simulink model "Y3Tiltrotor_sim3_IINDI_case2_1"  (R2025a)
settings: Solver=ode4  StartTime=0.0  StopTime=80  FixedStep=uavParam.sampleTime  RelTol=1e-3
PreLoadFcn:
  | filepath  = fileparts(get_param(bdroot, 'FileName'))
  | cd(filepath);
InitFcn:
  | Init_sim_IINDI_case2_1;
values from neighbouring files (symbols this model uses):
  a_HOD_p = 5    [Init_sim_IINDI_case2.m]    (also in Init_sim_IINDI_case2_1.m)
  a_HOD_q = 5    [Init_sim_IINDI_case2.m]    (also in Init_sim_IINDI_case2_1.m = 25)
  a_HOD_r = 5    [Init_sim_IINDI_case2.m]    (also in Init_sim_IINDI_case2_1.m)
  a_HOD_u = 5    [Init_sim_IINDI_case2.m]    (also in Init_sim_IINDI_case2_1.m = 15)
  a_HOD_v = 2    [Init_sim_IINDI_case2.m]    (also in Init_sim_IINDI_case2_1.m)
  a_HOD_w = 30    [Init_sim_IINDI_case2.m]    (also in Init_sim_IINDI_case2_1.m = 10)
  control = struct    [Init_sim_IINDI_case2.m]    (also in Init_sim_IINDI_case2_1.m)
  env = struct    [InitData.m]
  flightState = struct    [Init_sim_IINDI_case2.m]    (also in Init_sim_IINDI_case2_1.m)
  FWSpeed0 = 15    [Init_sim_IINDI_case2.m]    (also in Init_sim_IINDI_case2_1.m)
  k_lpf_p = 50    [Init_sim_IINDI_case2.m]    (also in Init_sim_IINDI_case2_1.m)
  k_lpf_q = 80    [Init_sim_IINDI_case2.m]    (also in Init_sim_IINDI_case2_1.m = 150)
  k_lpf_r = 100    [Init_sim_IINDI_case2.m]    (also in Init_sim_IINDI_case2_1.m)
  k_lpf_u = 8    [Init_sim_IINDI_case2.m]    (also in Init_sim_IINDI_case2_1.m)
  k_lpf_v = 1.5    [Init_sim_IINDI_case2.m]    (also in Init_sim_IINDI_case2_1.m)
  k_lpf_w = 50    [Init_sim_IINDI_case2.m]    (also in Init_sim_IINDI_case2_1.m)
  k_p = 5    [Init_sim_IINDI_case2.m]    (also in Init_sim_IINDI_case2_1.m)
  k_q = 12    [Init_sim_IINDI_case2.m]    (also in Init_sim_IINDI_case2_1.m)
  k_r = 0.1    [Init_sim_IINDI_case2.m]    (also in Init_sim_IINDI_case2_1.m)
  k_u = 0.2    [Init_sim_IINDI_case2.m]    (also in Init_sim_IINDI_case2_1.m = 1)
  k_v = 0.7    [Init_sim_IINDI_case2.m]    (also in Init_sim_IINDI_case2_1.m = 0.2)
  k_w = 2    [Init_sim_IINDI_case2.m]    (also in Init_sim_IINDI_case2_1.m)
  l_p = 30    [Init_sim_IINDI_case2.m]    (also in Init_sim_IINDI_case2_1.m)
  l_q = 15    [Init_sim_IINDI_case2.m]    (also in Init_sim_IINDI_case2_1.m)
  l_r = 25    [Init_sim_IINDI_case2.m]    (also in Init_sim_IINDI_case2_1.m)
  l_u = 1    [Init_sim_IINDI_case2.m]    (also in Init_sim_IINDI_case2_1.m = 0.8)
  l_v = 1.2    [Init_sim_IINDI_case2.m]    (also in Init_sim_IINDI_case2_1.m)
  l_w = 1    [Init_sim_IINDI_case2.m]    (also in Init_sim_IINDI_case2_1.m)
  lamda_p = 10    [Init_sim_IINDI_case2.m]    (also in Init_sim_IINDI_case2_1.m)
  lamda_q = 5    [Init_sim_IINDI_case2.m]    (also in Init_sim_IINDI_case2_1.m)
  lamda_r = 1    [Init_sim_IINDI_case2.m]    (also in Init_sim_IINDI_case2_1.m)
  lamda_u = 1    [Init_sim_IINDI_case2.m]    (also in Init_sim_IINDI_case2_1.m)
  lamda_v = 0.15    [Init_sim_IINDI_case2.m]    (also in Init_sim_IINDI_case2_1.m)
  lamda_w = 1    [Init_sim_IINDI_case2.m]    (also in Init_sim_IINDI_case2_1.m)
  uavParam = struct    [InitData.m]
undefined symbols (not defined in the file or in its folder): a_HOD, a_HOD_uvw, ControlSampleTime, F, Light, MIL, Newton, Raphson
libraries: slpidlib x31, SignalEditorBlockLib x15, simulink x3, aerolibtransform2 x3, sharedtransform x3, robotcorelib x3, matrix_library x3, aerolibasang x2, aerolibutil x2, aerolibwind2 x2, shared6dof x1, aerolibatmos2 x1
(part 2 of 8)

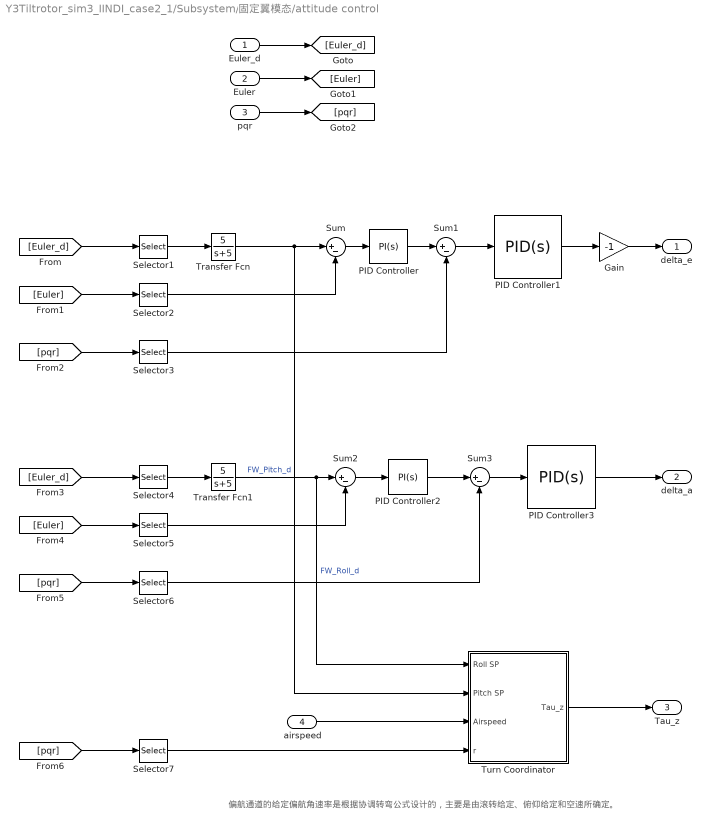
== system Y3Tiltrotor_sim3_IINDI_case2_1/Subsystem/固定翼模态/attitude control ==
  note: 偏航通道的给定偏航角速率是根据协调转弯公式设计的，主要是由滚转给定、俯仰给定和空速所确定。
  Euler_d : Inport
  Euler : Inport  Port=2
  pqr : Inport  Port=3
  airspeed : Inport  Port=4
  Gain : Gain  Gain=-1
  PID Controller : slpidlib/PID Controller  Controller=PI  Form=Parallel  TimeDomain=Continuous-time  UseExternalTs=off  SampleTime=ControlSampleTime  IntegratorMethod=Forward Euler  FilterMethod=Forward Euler  ControllerParametersSource=internal  P=control.FW.pitch_P  I=control.FW.pitch_I  UseKiTs=off  D=0  UseExternalDerivativeSource=off  N=100  UseFilter=on  TunerSelectOption=Transfer Function Based (PID Tuner App)  InitialConditionSource=internal  InitialConditionForIntegrator=0  InitialConditionForFilter=0  DifferentiatorICPrevScaledInput=0  ExternalReset=none  TrackingMode=off  Kt=1  LimitOutput=on  SatLimitsSource=internal  UpperSaturationLimit=control.maxPitchRate  LowerSaturationLimit=control.minPitchRate  LinearizeAsGain=on  AntiWindupMode=clamping  Kb=1  LimitIntegrator=off  UpperIntegratorSaturationLimit=inf  LowerIntegratorSaturationLimit=-inf  POutMin=[]  POutMax=[]  IOutMin=[]  IOutMax=[]  DOutMin=[]  DOutMax=[]  NOutMin=[]  NOutMax=[]  SumOutMin=[]  SumOutMax=[]  SaturationOutMin=[]  SaturationOutMax=[]  PParamMin=[]  PParamMax=[]  IParamMin=[]  IParamMax=[]  DParamMin=[]  DParamMax=[]  NParamMin=[]  NParamMax=[]  KbParamMin=[]  KbParamMax=[]  KtParamMin=[]  KtParamMax=[]  KbOutMin=[]  KbOutMax=[]  KtOutMin=[]  KtOutMax=[]  IntegratorOutMin=[]  IntegratorOutMax=[]  FilterOutMin=[]  FilterOutMax=[]  SumI1OutMin=[]  SumI1OutMax=[]  SumI2OutMin=[]  SumI2OutMax=[]  SumI3OutMin=[]  SumI3OutMax=[]  SumI4OutMin=[]  SumI4OutMax=[]  SumDOutMin=[]  SumDOutMax=[]  DifferentiatorOutMin=[]  DifferentiatorOutMax=[]  FilterDiffOutCoefMin=[]  FilterDiffOutCoefMax=[]  ReciprocalOutMin=[]  ReciprocalOutMax=[]  SumDenOutMin=[]  SumDenOutMax=[]  SumNumOutMin=[]  SumNumOutMax=[]  DivideOutMin=[]  DivideOutMax=[]  UdiffTsProdOutMin=[]  UdiffTsProdOutMax=[]  NTsProdOutMin=[]  NTsProdOutMax=[]  UintegralTsProdOutMin=[]  UintegralTsProdOutMax=[]  UngainTsProdOutMin=[]  UngainTsProdOutMax=[]  ClampingZeroOutDataTypeStr=Inherit: Inherit via back propagation  ClampingZeroOutMin=[]  ClampingZeroOutMax=[]  FilterDenConstantOutDataTypeStr=Inherit: Inherit via back propagation  FilterDenConstantOutMin=[]  FilterDenConstantOutMax=[]  PCopyOutDataTypeStr=Inherit: Inherit via back propagation  PCopyOutMin=[]  PCopyOutMax=[]  NCopyOutDataTypeStr=Inherit: Inherit via back propagation  NCopyOutMin=[]  NCopyOutMax=[]  IntegratorContinuousStateAttributes=''  IntegratorStateMustResolveToSignalObject=off  IntegratorRTWStateStorageClass=Auto  FilterContinuousStateAttributes=''  FilterStateMustResolveToSignalObject=off  FilterRTWStateStorageClass=Auto  ParallelPVariant=InternalParameters  IdealPVariant=Disabled  IVariant=InternalParameters  DVariant=Disabled  IntegratorVariant=Continuous  SatVariant=Enabled  AWVariant=ContClampingParallel  PCopyVariant=Disabled  TRVariant=Disabled  FdbkBlocksVariant=Forward  IdealPFdbkVariant=Disabled  SatFdbkVariant=Disabled  DerivativeFilterVariant=Disabled  NVariant=Disabled  NCopyVariant=Disabled_SignalSpec  FilterICVariant=Disabled  IntegratorICVariant=InternalICs  ExternalResetVariant=Disabled  TRSumVariant=Passthrough  SumFdbkVariant=Disabled  SumVariant=Sum_PI  TsampFilterVariant=InternalTs  TsampNgainVariant=Passthrough  TsampIntegralVariant=Disabled_SignalSpec  ExternalSaturationOutDataTypeStr=Inherit: Same as second input  DerivativeSourceVariant=Disabled  PreIntVariant=InternalPreInt
  PID Controller1 : slpidlib/PID Controller  Controller=PID  Form=Parallel  TimeDomain=Continuous-time  UseExternalTs=off  SampleTime=ControlSampleTime  IntegratorMethod=Forward Euler  FilterMethod=Forward Euler  ControllerParametersSource=internal  P=control.FW.pitchRate_P  I=control.FW.pitchRate_I  UseKiTs=off  D=control.FW.pitchRate_D  UseExternalDerivativeSource=off  N=10  UseFilter=on  TunerSelectOption=Transfer Function Based (PID Tuner App)  InitialConditionSource=internal  InitialConditionForIntegrator=0  InitialConditionForFilter=0  DifferentiatorICPrevScaledInput=0  ExternalReset=none  TrackingMode=off  Kt=1  LimitOutput=on  SatLimitsSource=internal  UpperSaturationLimit=pi/2  LowerSaturationLimit=-pi/2  LinearizeAsGain=on  AntiWindupMode=clamping  Kb=1  LimitIntegrator=off  UpperIntegratorSaturationLimit=inf  LowerIntegratorSaturationLimit=-inf  POutMin=[]  POutMax=[]  IOutMin=[]  IOutMax=[]  DOutMin=[]  DOutMax=[]  NOutMin=[]  NOutMax=[]  SumOutMin=[]  SumOutMax=[]  SaturationOutMin=[]  SaturationOutMax=[]  PParamMin=[]  PParamMax=[]  IParamMin=[]  IParamMax=[]  DParamMin=[]  DParamMax=[]  NParamMin=[]  NParamMax=[]  KbParamMin=[]  KbParamMax=[]  KtParamMin=[]  KtParamMax=[]  KbOutMin=[]  KbOutMax=[]  KtOutMin=[]  KtOutMax=[]  IntegratorOutMin=[]  IntegratorOutMax=[]  FilterOutMin=[]  FilterOutMax=[]  SumI1OutMin=[]  SumI1OutMax=[]  SumI2OutMin=[]  SumI2OutMax=[]  SumI3OutMin=[]  SumI3OutMax=[]  SumI4OutMin=[]  SumI4OutMax=[]  SumDOutMin=[]  SumDOutMax=[]  DifferentiatorOutMin=[]  DifferentiatorOutMax=[]  FilterDiffOutCoefMin=[]  FilterDiffOutCoefMax=[]  ReciprocalOutMin=[]  ReciprocalOutMax=[]  SumDenOutMin=[]  SumDenOutMax=[]  SumNumOutMin=[]  SumNumOutMax=[]  DivideOutMin=[]  DivideOutMax=[]  UdiffTsProdOutMin=[]  UdiffTsProdOutMax=[]  NTsProdOutMin=[]  NTsProdOutMax=[]  UintegralTsProdOutMin=[]  UintegralTsProdOutMax=[]  UngainTsProdOutMin=[]  UngainTsProdOutMax=[]  ClampingZeroOutDataTypeStr=Inherit: Inherit via back propagation  ClampingZeroOutMin=[]  ClampingZeroOutMax=[]  FilterDenConstantOutDataTypeStr=Inherit: Inherit via back propagation  FilterDenConstantOutMin=[]  FilterDenConstantOutMax=[]  PCopyOutDataTypeStr=Inherit: Inherit via back propagation  PCopyOutMin=[]  PCopyOutMax=[]  NCopyOutDataTypeStr=Inherit: Inherit via back propagation  NCopyOutMin=[]  NCopyOutMax=[]  IntegratorContinuousStateAttributes=''  IntegratorStateMustResolveToSignalObject=off  IntegratorRTWStateStorageClass=Auto  FilterContinuousStateAttributes=''  FilterStateMustResolveToSignalObject=off  FilterRTWStateStorageClass=Auto  ParallelPVariant=InternalParameters  IdealPVariant=Disabled  IVariant=InternalParameters  DVariant=InternalParameters  IntegratorVariant=Continuous  SatVariant=Enabled  AWVariant=ContClampingParallel  PCopyVariant=Disabled  TRVariant=Disabled  FdbkBlocksVariant=Forward  IdealPFdbkVariant=Disabled  SatFdbkVariant=Disabled  DerivativeFilterVariant=ContFilter  NVariant=InternalParameters  NCopyVariant=Disabled  FilterICVariant=InternalICsFilter  IntegratorICVariant=InternalICs  ExternalResetVariant=Disabled  TRSumVariant=Passthrough  SumFdbkVariant=Disabled  SumVariant=Sum_PID  TsampFilterVariant=InternalTs  TsampNgainVariant=Passthrough  TsampIntegralVariant=Disabled_SignalSpec  ExternalSaturationOutDataTypeStr=Inherit: Same as second input  DerivativeSourceVariant=ErrorSignal  PreIntVariant=InternalPreInt
  PID Controller2 : slpidlib/PID Controller  Controller=PI  Form=Parallel  TimeDomain=Continuous-time  UseExternalTs=off  SampleTime=ControlSampleTime  IntegratorMethod=Forward Euler  FilterMethod=Forward Euler  ControllerParametersSource=internal  P=control.FW.roll_P  I=control.FW.roll_I  UseKiTs=off  D=0  UseExternalDerivativeSource=off  N=100  UseFilter=on  TunerSelectOption=Transfer Function Based (PID Tuner App)  InitialConditionSource=internal  InitialConditionForIntegrator=0  InitialConditionForFilter=0  DifferentiatorICPrevScaledInput=0  ExternalReset=none  TrackingMode=off  Kt=1  LimitOutput=on  SatLimitsSource=internal  UpperSaturationLimit=control.maxRollRate  LowerSaturationLimit=control.minRollRate  LinearizeAsGain=on  AntiWindupMode=clamping  Kb=1  LimitIntegrator=off  UpperIntegratorSaturationLimit=inf  LowerIntegratorSaturationLimit=-inf  POutMin=[]  POutMax=[]  IOutMin=[]  IOutMax=[]  DOutMin=[]  DOutMax=[]  NOutMin=[]  NOutMax=[]  SumOutMin=[]  SumOutMax=[]  SaturationOutMin=[]  SaturationOutMax=[]  PParamMin=[]  PParamMax=[]  IParamMin=[]  IParamMax=[]  DParamMin=[]  DParamMax=[]  NParamMin=[]  NParamMax=[]  KbParamMin=[]  KbParamMax=[]  KtParamMin=[]  KtParamMax=[]  KbOutMin=[]  KbOutMax=[]  KtOutMin=[]  KtOutMax=[]  IntegratorOutMin=[]  IntegratorOutMax=[]  FilterOutMin=[]  FilterOutMax=[]  SumI1OutMin=[]  SumI1OutMax=[]  SumI2OutMin=[]  SumI2OutMax=[]  SumI3OutMin=[]  SumI3OutMax=[]  SumI4OutMin=[]  SumI4OutMax=[]  SumDOutMin=[]  SumDOutMax=[]  DifferentiatorOutMin=[]  DifferentiatorOutMax=[]  FilterDiffOutCoefMin=[]  FilterDiffOutCoefMax=[]  ReciprocalOutMin=[]  ReciprocalOutMax=[]  SumDenOutMin=[]  SumDenOutMax=[]  SumNumOutMin=[]  SumNumOutMax=[]  DivideOutMin=[]  DivideOutMax=[]  UdiffTsProdOutMin=[]  UdiffTsProdOutMax=[]  NTsProdOutMin=[]  NTsProdOutMax=[]  UintegralTsProdOutMin=[]  UintegralTsProdOutMax=[]  UngainTsProdOutMin=[]  UngainTsProdOutMax=[]  ClampingZeroOutDataTypeStr=Inherit: Inherit via back propagation  ClampingZeroOutMin=[]  ClampingZeroOutMax=[]  FilterDenConstantOutDataTypeStr=Inherit: Inherit via back propagation  FilterDenConstantOutMin=[]  FilterDenConstantOutMax=[]  PCopyOutDataTypeStr=Inherit: Inherit via back propagation  PCopyOutMin=[]  PCopyOutMax=[]  NCopyOutDataTypeStr=Inherit: Inherit via back propagation  NCopyOutMin=[]  NCopyOutMax=[]  IntegratorContinuousStateAttributes=''  IntegratorStateMustResolveToSignalObject=off  IntegratorRTWStateStorageClass=Auto  FilterContinuousStateAttributes=''  FilterStateMustResolveToSignalObject=off  FilterRTWStateStorageClass=Auto  ParallelPVariant=InternalParameters  IdealPVariant=Disabled  IVariant=InternalParameters  DVariant=Disabled  IntegratorVariant=Continuous  SatVariant=Enabled  AWVariant=ContClampingParallel  PCopyVariant=Disabled  TRVariant=Disabled  FdbkBlocksVariant=Forward  IdealPFdbkVariant=Disabled  SatFdbkVariant=Disabled  DerivativeFilterVariant=Disabled  NVariant=Disabled  NCopyVariant=Disabled_SignalSpec  FilterICVariant=Disabled  IntegratorICVariant=InternalICs  ExternalResetVariant=Disabled  TRSumVariant=Passthrough  SumFdbkVariant=Disabled  SumVariant=Sum_PI  TsampFilterVariant=InternalTs  TsampNgainVariant=Passthrough  TsampIntegralVariant=Disabled_SignalSpec  ExternalSaturationOutDataTypeStr=Inherit: Same as second input  DerivativeSourceVariant=Disabled  PreIntVariant=InternalPreInt
  PID Controller3 : slpidlib/PID Controller  Controller=PID  Form=Parallel  TimeDomain=Continuous-time  UseExternalTs=off  SampleTime=ControlSampleTime  IntegratorMethod=Forward Euler  FilterMethod=Forward Euler  ControllerParametersSource=internal  P=control.FW.rollRate_P  I=control.FW.rollRate_I  UseKiTs=off  D=control.FW.rollRate_D  UseExternalDerivativeSource=off  N=10  UseFilter=on  TunerSelectOption=Transfer Function Based (PID Tuner App)  InitialConditionSource=internal  InitialConditionForIntegrator=0  InitialConditionForFilter=0  DifferentiatorICPrevScaledInput=0  ExternalReset=none  TrackingMode=off  Kt=1  LimitOutput=on  SatLimitsSource=internal  UpperSaturationLimit=pi/2  LowerSaturationLimit=-pi/2  LinearizeAsGain=on  AntiWindupMode=clamping  Kb=1  LimitIntegrator=off  UpperIntegratorSaturationLimit=inf  LowerIntegratorSaturationLimit=-inf  POutMin=[]  POutMax=[]  IOutMin=[]  IOutMax=[]  DOutMin=[]  DOutMax=[]  NOutMin=[]  NOutMax=[]  SumOutMin=[]  SumOutMax=[]  SaturationOutMin=[]  SaturationOutMax=[]  PParamMin=[]  PParamMax=[]  IParamMin=[]  IParamMax=[]  DParamMin=[]  DParamMax=[]  NParamMin=[]  NParamMax=[]  KbParamMin=[]  KbParamMax=[]  KtParamMin=[]  KtParamMax=[]  KbOutMin=[]  KbOutMax=[]  KtOutMin=[]  KtOutMax=[]  IntegratorOutMin=[]  IntegratorOutMax=[]  FilterOutMin=[]  FilterOutMax=[]  SumI1OutMin=[]  SumI1OutMax=[]  SumI2OutMin=[]  SumI2OutMax=[]  SumI3OutMin=[]  SumI3OutMax=[]  SumI4OutMin=[]  SumI4OutMax=[]  SumDOutMin=[]  SumDOutMax=[]  DifferentiatorOutMin=[]  DifferentiatorOutMax=[]  FilterDiffOutCoefMin=[]  FilterDiffOutCoefMax=[]  ReciprocalOutMin=[]  ReciprocalOutMax=[]  SumDenOutMin=[]  SumDenOutMax=[]  SumNumOutMin=[]  SumNumOutMax=[]  DivideOutMin=[]  DivideOutMax=[]  UdiffTsProdOutMin=[]  UdiffTsProdOutMax=[]  NTsProdOutMin=[]  NTsProdOutMax=[]  UintegralTsProdOutMin=[]  UintegralTsProdOutMax=[]  UngainTsProdOutMin=[]  UngainTsProdOutMax=[]  ClampingZeroOutDataTypeStr=Inherit: Inherit via back propagation  ClampingZeroOutMin=[]  ClampingZeroOutMax=[]  FilterDenConstantOutDataTypeStr=Inherit: Inherit via back propagation  FilterDenConstantOutMin=[]  FilterDenConstantOutMax=[]  PCopyOutDataTypeStr=Inherit: Inherit via back propagation  PCopyOutMin=[]  PCopyOutMax=[]  NCopyOutDataTypeStr=Inherit: Inherit via back propagation  NCopyOutMin=[]  NCopyOutMax=[]  IntegratorContinuousStateAttributes=''  IntegratorStateMustResolveToSignalObject=off  IntegratorRTWStateStorageClass=Auto  FilterContinuousStateAttributes=''  FilterStateMustResolveToSignalObject=off  FilterRTWStateStorageClass=Auto  ParallelPVariant=InternalParameters  IdealPVariant=Disabled  IVariant=InternalParameters  DVariant=InternalParameters  IntegratorVariant=Continuous  SatVariant=Enabled  AWVariant=ContClampingParallel  PCopyVariant=Disabled  TRVariant=Disabled  FdbkBlocksVariant=Forward  IdealPFdbkVariant=Disabled  SatFdbkVariant=Disabled  DerivativeFilterVariant=ContFilter  NVariant=InternalParameters  NCopyVariant=Disabled  FilterICVariant=InternalICsFilter  IntegratorICVariant=InternalICs  ExternalResetVariant=Disabled  TRSumVariant=Passthrough  SumFdbkVariant=Disabled  SumVariant=Sum_PID  TsampFilterVariant=InternalTs  TsampNgainVariant=Passthrough  TsampIntegralVariant=Disabled_SignalSpec  ExternalSaturationOutDataTypeStr=Inherit: Same as second input  DerivativeSourceVariant=ErrorSignal  PreIntVariant=InternalPreInt
  Selector1 : Selector  InputPortWidth=3  IndexOptions=Index vector (dialog)  Indices=2  OutputSizes=1
  Selector2 : Selector  InputPortWidth=3  IndexOptions=Index vector (dialog)  Indices=2  OutputSizes=1
  Selector3 : Selector  InputPortWidth=3  IndexOptions=Index vector (dialog)  Indices=2  OutputSizes=1
  Selector4 : Selector  InputPortWidth=3  IndexOptions=Index vector (dialog)  Indices=1  OutputSizes=1
  Selector5 : Selector  InputPortWidth=3  IndexOptions=Index vector (dialog)  Indices=1  OutputSizes=1
  Selector6 : Selector  InputPortWidth=3  IndexOptions=Index vector (dialog)  Indices=1  OutputSizes=1
  Selector7 : Selector  InputPortWidth=3  IndexOptions=Index vector (dialog)  Indices=3  OutputSizes=1
  Sum{,1..3} (4 alike) : Sum  Inputs=|+-
  Transfer Fcn : TransferFcn  Numerator=[5]  Denominator=[1 5]
  Transfer Fcn1 : TransferFcn  Numerator=[5]  Denominator=[1 5]
  Turn Coordinator : Subsystem
  delta_e : Outport
  delta_a : Outport  Port=2
  Tau_z : Outport  Port=3
  wires:
  Selector2/1 -> Sum/2
  Sum/1 -> PID Controller/1
  Selector3/1 -> Sum1/2
  Sum1/1 -> PID Controller1/1
  PID Controller1/1 -> Gain/1
  Selector1/1 -> Transfer Fcn/1
  PID Controller/1 -> Sum1/1
  Euler_d/1 -> [Euler_d]
  Euler/1 -> [Euler]
  pqr/1 -> [pqr]
  [Euler_d] -> Selector1/1
  [Euler] -> Selector2/1
  [pqr] -> Selector3/1
  [pqr] -> Selector6/1
  [Euler_d] -> Selector4/1
  [Euler] -> Selector5/1
  Transfer Fcn1/1 -> Turn Coordinator/1(Roll SP), Sum2/1  "FW_Roll_d"
  Selector5/1 -> Sum2/2
  Sum2/1 -> PID Controller2/1
  Sum3/1 -> PID Controller3/1
  Selector6/1 -> Sum3/2
  PID Controller2/1 -> Sum3/1
  Selector4/1 -> Transfer Fcn1/1
  airspeed/1 -> Turn Coordinator/3(Airspeed)
  [pqr] -> Selector7/1
  Selector7/1 -> Turn Coordinator/4(r)
  Transfer Fcn/1 -> Turn Coordinator/2(Pitch SP), Sum/1  "FW_Pitch_d"
  Gain/1 -> delta_e/1
  PID Controller3/1 -> delta_a/1
  Turn Coordinator/1(Tau_z) -> Tau_z/1

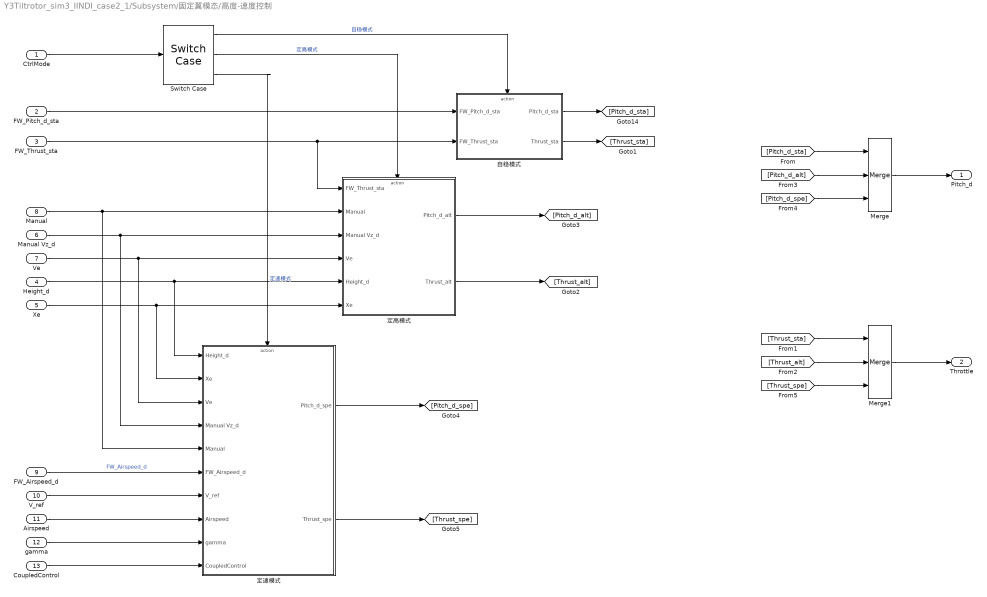
== system Y3Tiltrotor_sim3_IINDI_case2_1/Subsystem/固定翼模态/高度-速度控制 ==
  CtrlMode : Inport
  FW_Pitch_d_sta : Inport  Port=2
  FW_Thrust_sta : Inport  Port=3
  Height_d : Inport  Port=4
  Xe : Inport  Port=5
  Manual Vz_d : Inport  Port=6
  Ve : Inport  Port=7
  Manual : Inport  Port=8
  FW_Airspeed_d : Inport  Port=9
  V_ref : Inport  Port=10
  Airspeed : Inport  Port=11
  gamma : Inport  Port=12
  CoupledControl : Inport  Port=13
  Merge : Merge  Inputs=3
  Merge1 : Merge  Inputs=3
  Switch Case : SwitchCase  CaseConditions={0,1,2}  ShowDefaultCase=off
  定速模式 : Subsystem
  定高模式 : Subsystem
  自稳模式 : Subsystem
  Pitch_d : Outport
  Throttle : Outport  Port=2
  wires:
  Switch Case/3 -> 定速模式/Action  "定速模式"
  Switch Case/1 -> 自稳模式/Action  "自稳模式"
  Switch Case/2 -> 定高模式/Action  "定高模式"
  CtrlMode/1 -> Switch Case/1
  FW_Pitch_d_sta/1 -> 自稳模式/1(FW_Pitch_d_sta)
  FW_Thrust_sta/1 -> 定高模式/1(FW_Thrust_sta), 自稳模式/2(FW_Thrust_sta)
  Merge/1 -> Pitch_d/1
  自稳模式/1(Pitch_d_sta) -> [Pitch_d_sta]
  自稳模式/2(Thrust_sta) -> [Thrust_sta]
  [Pitch_d_sta] -> Merge/1
  [Thrust_sta] -> Merge1/1
  定高模式/2(Thrust_alt) -> [Thrust_alt]
  [Thrust_alt] -> Merge1/2
  定高模式/1(Pitch_d_alt) -> [Pitch_d_alt]
  Xe/1 -> 定速模式/2(Xe), 定高模式/6(Xe)
  Manual Vz_d/1 -> 定速模式/4(Manual Vz_d), 定高模式/3(Manual Vz_d)
  Ve/1 -> 定速模式/3(Ve), 定高模式/4(Ve)
  Manual/1 -> 定高模式/2(Manual), 定速模式/5(Manual)
  定速模式/1(Pitch_d_spe) -> [Pitch_d_spe]
  定速模式/2(Thrust_spe) -> [Thrust_spe]
  [Pitch_d_spe] -> Merge/3
  [Thrust_spe] -> Merge1/3
  Height_d/1 -> 定速模式/1(Height_d), 定高模式/5(Height_d)
  FW_Airspeed_d/1 -> 定速模式/6(FW_Airspeed_d)  "FW_Airspeed_d"
  Airspeed/1 -> 定速模式/8(Airspeed)
  gamma/1 -> 定速模式/9(gamma)
  CoupledControl/1 -> 定速模式/10(CoupledControl)
  [Pitch_d_alt] -> Merge/2
  V_ref/1 -> 定速模式/7(V_ref)
  Merge1/1 -> Throttle/1

== system Y3Tiltrotor_sim3_IINDI_case2_1/Subsystem/多旋翼模态/InputConditioning_stablelize ==
  Ch1 : Inport
  Ch2 : Inport  Port=2
  Ch3 : Inport  Port=3
  Ch4 : Inport  Port=4
  Manual : Inport  Port=5
  theta_ref : Inport  Port=6
  Constant : Constant
  Constant1 : Constant  Value=0
  Gain : Gain  Gain=0.5
  Gain13 : Gain  Gain=control.maxPitch
  Gain14 : Gain  Gain=control.maxRoll
  Gain15 : Gain  Gain=control.maxYawRate
  Gain16 : Gain  Gain=3
  Gain2 : Gain  Gain=pi/180
  Saturation{1,7..9} (4 alike) : Saturate  UpperLimit=1  LowerLimit=-1
  Saturation10 : Saturate  UpperLimit=1  LowerLimit=0
  Saturation4 : Saturate  UpperLimit=3  LowerLimit=0
  Sum : Sum  Inputs=|++
  Switch : Switch  Criteria=u2 > Threshold  SaturateOnIntegerOverflow=off  InputSameDT=off
  deadzone0 : MATLAB Function  TreatAsAtomicUnit=on
  deadzone1 : MATLAB Function  TreatAsAtomicUnit=on
  deadzone2 : MATLAB Function  TreatAsAtomicUnit=on
  deadzone3 : MATLAB Function  TreatAsAtomicUnit=on
  pitch_d1 : SignalEditorBlockLib/Signal Editor  FileName=pitch_d.mat  ActiveScenario=Test  ActiveSignal=俯仰角测试-遥控器  IsBus=off  OutputBusObjectStr=Bus: BusObject  SampleTime=0  ZeroCross=off  OutputAfterFinalValue=Setting to zero  Unit=inherit  PreserveSignalName=on  ApplySigPropsToAllScenarios=on  ApplySigPropsToAllSignals=on  SignalPropertySource=Dialog parameters
  Roll_cmd : Outport  VectorParamsAs1DForOutWhenUnconnected=off
  Pitch_cmd : Outport  Port=2  VectorParamsAs1DForOutWhenUnconnected=off
  YawRate_cmd : Outport  Port=3  VectorParamsAs1DForOutWhenUnconnected=off
  Thrust_cmd : Outport  Port=4  VectorParamsAs1DForOutWhenUnconnected=off
  wires:
  Saturation10/1 -> Gain16/1
  Saturation7/1 -> Gain15/1
  Saturation9/1 -> Gain14/1
  Saturation8/1 -> Gain13/1
  deadzone0/1(y) -> Saturation9/1
  deadzone1/1(y) -> Saturation8/1
  deadzone2/1(y) -> Saturation7/1
  Ch1/1 -> deadzone1/1(u)
  Ch3/1 -> deadzone3/1(u)
  Ch2/1 -> deadzone0/1(u)
  Ch4/1 -> deadzone2/1(u)
  deadzone3/1(y) -> Saturation1/1
  Sum/1 -> Gain/1
  Saturation1/1 -> Sum/1
  Gain/1 -> Saturation10/1
  Constant/1 -> Sum/2
  Gain14/1 -> Roll_cmd/1
  Gain15/1 -> YawRate_cmd/1
  Gain16/1 -> Saturation4/1
  Saturation4/1 -> Thrust_cmd/1  "Throttle_sat"
  Manual/1 -> Switch/2
  theta_ref/1 -> Switch/3
  Gain13/1 -> Switch/1
  ? -> Gain2/1
  Switch/1 -> Pitch_cmd/1

== system Y3Tiltrotor_sim3_IINDI_case2_1/Subsystem/多旋翼模态/Multirotor XY control ==
  note: 前向通道控制
  note: 横侧向通道控制
  x_ref : Inport
  y_ref : Inport  Port=2
  xe : Inport  Port=3
  Ch8 : Inport  Port=4
  Ch2 : Inport  Port=5
  Manual : Inport  Port=6
  Selector1 : Selector  InputPortWidth=3  IndexOptions=Index vector (dialog)  Indices=2  OutputSizes=1
  Selector6 : Selector  InputPortWidth=3  IndexOptions=Index vector (dialog)  Indices=1  OutputSizes=1
  Subsystem : Subsystem
  Subsystem3 : Subsystem
  MR_vx_d : Outport
  MR_vy_d : Outport  Port=2
  wires:
  Subsystem3/1(MR_vx_d) -> MR_vx_d/1
  y_ref/1 -> Subsystem/4(y_ref)
  Ch2/1 -> Subsystem/3(Ch2)
  Manual/1 -> [Manual]
  [Manual] -> Subsystem/2(Manual)
  Subsystem/1(MR_vy_d) -> MR_vy_d/1
  [Manual] -> Subsystem3/1(Manual)
  Ch8/1 -> Subsystem3/2(Ch8)
  x_ref/1 -> Subsystem3/3(x_ref)
  Selector6/1 -> Subsystem3/4(x)
  xe/1 -> Selector6/1, Selector1/1
  Selector1/1 -> Subsystem/1(y)

== system Y3Tiltrotor_sim3_IINDI_case2_1/Subsystem/多旋翼模态/Multirotor XY control1 ==
  note: 前向通道控制
  note: 横侧向通道控制
  ex : Inport
  ey : Inport  Port=2
  ez : Inport  Port=3
  Ch8 : Inport  Port=4
  Ch2 : Inport  Port=5
  Manual : Inport  Port=6
  DCMbe : Inport  Port=7
  Subsystem : Subsystem
  Subsystem3 : Subsystem
  Transfer Fcn : TransferFcn  Numerator=[4]  Denominator=[1 4]
  Transfer Fcn1 : TransferFcn  Numerator=[4]  Denominator=[1 4]
  MR_vfor_d : Outport
  MR_vlat_d : Outport  Port=2
  wires:
  Subsystem3/1(MR_vfor_d) -> MR_vfor_d/1  "MR_vfor_d"
  [ex] -> Subsystem/3(ex)
  [ey] -> Subsystem/4(ey)
  Ch2/1 -> Subsystem/2(Ch2)
  Manual/1 -> [Manual]
  [Manual] -> Subsystem/1(Manual)
  Subsystem/1(MR_vlat_d) -> MR_vlat_d/1  "MR_vlat_d"
  [Manual] -> Subsystem3/1(Manual)
  Ch8/1 -> Subsystem3/2(Ch8)
  DCMbe/1 -> [DCMbe]
  [DCMbe] -> Subsystem/6(DCMbe)
  [ez] -> Subsystem/5(ez)
  [ex] -> Subsystem3/3(ex)
  [ey] -> Subsystem3/4(ey)
  [ez] -> Subsystem3/5(ez)
  [DCMbe] -> Subsystem3/6(DCMbe)
  ez/1 -> [ez]
  ex/1 -> [ex]
  ey/1 -> [ey]
  Transfer Fcn/1 -> ?
  Transfer Fcn1/1 -> ?

== system Y3Tiltrotor_sim3_IINDI_case2_1/Subsystem/多旋翼模态/Multirotor altitude control ==
  Manual : Inport
  Ch3 : Inport  Port=2
  Xe : Inport  Port=3
  z_ref : Inport  Port=4
  Gain : Gain  Gain=-1
  Subsystem : Subsystem
  Terminator : Terminator
  vz_d : Outport
  wires:
  Gain/1 -> Terminator/1  "MR_vz_d"
  Subsystem/1(vz_d) -> vz_d/1, Gain/1
  Ch3/1 -> Subsystem/2(Ch3)
  Xe/1 -> Subsystem/3(Xe)
  Manual/1 -> Subsystem/1(Manual)
  z_ref/1 -> Subsystem/4(z_ref)

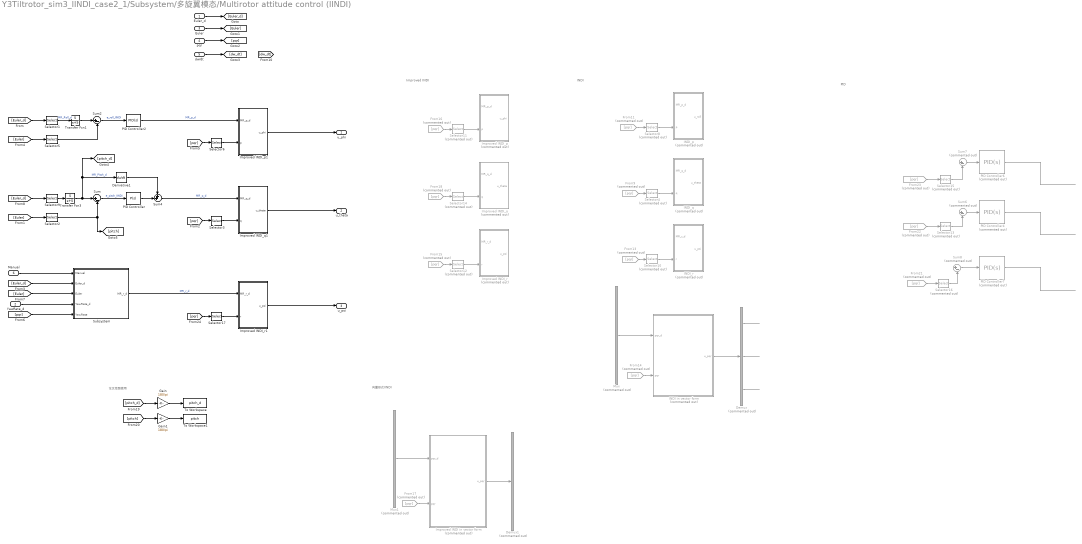
== system Y3Tiltrotor_sim3_IINDI_case2_1/Subsystem/多旋翼模态/Multirotor attitude control (IINDI) ==
  note: 论文绘图使用
  note: 向量形式IINDI
  note: Improved INDI
  note: INDI
  note: PID
  Euler_d : Inport
  YawRate_d : Inport  Port=2
  Euler : Inport  Port=3
  pqr : Inport  Port=4
  dw/dt : Inport  Port=5
  Manual : Inport  Port=6
  Demux : Demux  Commented=on  Outputs=3
  Demux1 : Demux  Commented=on  Outputs=3
  Derivative1 : Derivative
  From{9,11,13..18,21..23} (11 alike) : From  Commented=on  GotoTag=pqr
  Gain : Gain  Gain=180/pi
  Gain1 : Gain  Gain=180/pi
  INDI in vector form : Subsystem  Commented=on
  INDI_p : Subsystem  Commented=on
  INDI_q : Subsystem  Commented=on
  INDI_r : Subsystem  Commented=on
  Improved INDI in vector form : Subsystem  Commented=on
  Improved INDI_p : Subsystem  Commented=on
  Improved INDI_p1 : Subsystem
  Improved INDI_q : Subsystem  Commented=on
  Improved INDI_q1 : Subsystem
  Improved INDI_r : Subsystem  Commented=on
  Improved INDI_r1 : Subsystem
  Mux : Mux  Commented=on  Inputs=3
  Mux1 : Mux  Commented=on  Inputs=3
  PID Controller : slpidlib/PID Controller  Controller=P  Form=Parallel  TimeDomain=Continuous-time  UseExternalTs=off  SampleTime=ControlSampleTime  IntegratorMethod=Forward Euler  FilterMethod=Forward Euler  ControllerParametersSource=internal  P=control.MR.pitch_P  I=control.FW.pitch_I  UseKiTs=off  D=0  UseExternalDerivativeSource=off  N=100  UseFilter=on  TunerSelectOption=Transfer Function Based (PID Tuner App)  InitialConditionSource=internal  InitialConditionForIntegrator=0  InitialConditionForFilter=0  DifferentiatorICPrevScaledInput=0  ExternalReset=none  TrackingMode=off  Kt=1  LimitOutput=off  SatLimitsSource=internal  UpperSaturationLimit=control.maxPitchRate  LowerSaturationLimit=control.minPitchRate  LinearizeAsGain=on  AntiWindupMode=clamping  Kb=1  LimitIntegrator=off  UpperIntegratorSaturationLimit=inf  LowerIntegratorSaturationLimit=-inf  POutMin=[]  POutMax=[]  IOutMin=[]  IOutMax=[]  DOutMin=[]  DOutMax=[]  NOutMin=[]  NOutMax=[]  SumOutMin=[]  SumOutMax=[]  SaturationOutMin=[]  SaturationOutMax=[]  PParamMin=[]  PParamMax=[]  IParamMin=[]  IParamMax=[]  DParamMin=[]  DParamMax=[]  NParamMin=[]  NParamMax=[]  KbParamMin=[]  KbParamMax=[]  KtParamMin=[]  KtParamMax=[]  KbOutMin=[]  KbOutMax=[]  KtOutMin=[]  KtOutMax=[]  IntegratorOutMin=[]  IntegratorOutMax=[]  FilterOutMin=[]  FilterOutMax=[]  SumI1OutMin=[]  SumI1OutMax=[]  SumI2OutMin=[]  SumI2OutMax=[]  SumI3OutMin=[]  SumI3OutMax=[]  SumI4OutMin=[]  SumI4OutMax=[]  SumDOutMin=[]  SumDOutMax=[]  DifferentiatorOutMin=[]  DifferentiatorOutMax=[]  FilterDiffOutCoefMin=[]  FilterDiffOutCoefMax=[]  ReciprocalOutMin=[]  ReciprocalOutMax=[]  SumDenOutMin=[]  SumDenOutMax=[]  SumNumOutMin=[]  SumNumOutMax=[]  DivideOutMin=[]  DivideOutMax=[]  UdiffTsProdOutMin=[]  UdiffTsProdOutMax=[]  NTsProdOutMin=[]  NTsProdOutMax=[]  UintegralTsProdOutMin=[]  UintegralTsProdOutMax=[]  UngainTsProdOutMin=[]  UngainTsProdOutMax=[]  ClampingZeroOutDataTypeStr=Inherit: Inherit via back propagation  ClampingZeroOutMin=[]  ClampingZeroOutMax=[]  FilterDenConstantOutDataTypeStr=Inherit: Inherit via back propagation  FilterDenConstantOutMin=[]  FilterDenConstantOutMax=[]  PCopyOutDataTypeStr=Inherit: Inherit via back propagation  PCopyOutMin=[]  PCopyOutMax=[]  NCopyOutDataTypeStr=Inherit: Inherit via back propagation  NCopyOutMin=[]  NCopyOutMax=[]  IntegratorContinuousStateAttributes=''  IntegratorStateMustResolveToSignalObject=off  IntegratorRTWStateStorageClass=Auto  FilterContinuousStateAttributes=''  FilterStateMustResolveToSignalObject=off  FilterRTWStateStorageClass=Auto  ParallelPVariant=InternalParameters  IdealPVariant=Disabled  IVariant=Disabled  DVariant=Disabled  IntegratorVariant=Disabled  SatVariant=Disabled  AWVariant=Disabled  PCopyVariant=Disabled  TRVariant=Disabled  FdbkBlocksVariant=Forward  IdealPFdbkVariant=Disabled  SatFdbkVariant=Disabled  DerivativeFilterVariant=Disabled  NVariant=Disabled  NCopyVariant=Disabled_SignalSpec  FilterICVariant=Disabled  IntegratorICVariant=Disabled  ExternalResetVariant=Disabled  TRSumVariant=Passthrough  SumFdbkVariant=Disabled  SumVariant=Passthrough_P  TsampFilterVariant=InternalTs  TsampNgainVariant=Passthrough  TsampIntegralVariant=Disabled_SignalSpec  ExternalSaturationOutDataTypeStr=Inherit: Same as second input  DerivativeSourceVariant=Disabled  PreIntVariant=InternalPreInt
  PID Controller2 : slpidlib/PID Controller  Controller=PID  Form=Parallel  TimeDomain=Continuous-time  UseExternalTs=off  SampleTime=ControlSampleTime  IntegratorMethod=Forward Euler  FilterMethod=Forward Euler  ControllerParametersSource=internal  P=control.MR.roll_P  I=control.MR.roll_I  UseKiTs=off  D=control.MR.roll_D  UseExternalDerivativeSource=off  N=100  UseFilter=on  TunerSelectOption=Transfer Function Based (PID Tuner App)  InitialConditionSource=internal  InitialConditionForIntegrator=0  InitialConditionForFilter=0  DifferentiatorICPrevScaledInput=0  ExternalReset=none  TrackingMode=off  Kt=1  LimitOutput=off  SatLimitsSource=internal  UpperSaturationLimit=control.maxRollRate  LowerSaturationLimit=control.minRollRate  LinearizeAsGain=on  AntiWindupMode=clamping  Kb=1  LimitIntegrator=off  UpperIntegratorSaturationLimit=inf  LowerIntegratorSaturationLimit=-inf  POutMin=[]  POutMax=[]  IOutMin=[]  IOutMax=[]  DOutMin=[]  DOutMax=[]  NOutMin=[]  NOutMax=[]  SumOutMin=[]  SumOutMax=[]  SaturationOutMin=[]  SaturationOutMax=[]  PParamMin=[]  PParamMax=[]  IParamMin=[]  IParamMax=[]  DParamMin=[]  DParamMax=[]  NParamMin=[]  NParamMax=[]  KbParamMin=[]  KbParamMax=[]  KtParamMin=[]  KtParamMax=[]  KbOutMin=[]  KbOutMax=[]  KtOutMin=[]  KtOutMax=[]  IntegratorOutMin=[]  IntegratorOutMax=[]  FilterOutMin=[]  FilterOutMax=[]  SumI1OutMin=[]  SumI1OutMax=[]  SumI2OutMin=[]  SumI2OutMax=[]  SumI3OutMin=[]  SumI3OutMax=[]  SumI4OutMin=[]  SumI4OutMax=[]  SumDOutMin=[]  SumDOutMax=[]  DifferentiatorOutMin=[]  DifferentiatorOutMax=[]  FilterDiffOutCoefMin=[]  FilterDiffOutCoefMax=[]  ReciprocalOutMin=[]  ReciprocalOutMax=[]  SumDenOutMin=[]  SumDenOutMax=[]  SumNumOutMin=[]  SumNumOutMax=[]  DivideOutMin=[]  DivideOutMax=[]  UdiffTsProdOutMin=[]  UdiffTsProdOutMax=[]  NTsProdOutMin=[]  NTsProdOutMax=[]  UintegralTsProdOutMin=[]  UintegralTsProdOutMax=[]  UngainTsProdOutMin=[]  UngainTsProdOutMax=[]  ClampingZeroOutDataTypeStr=Inherit: Inherit via back propagation  ClampingZeroOutMin=[]  ClampingZeroOutMax=[]  FilterDenConstantOutDataTypeStr=Inherit: Inherit via back propagation  FilterDenConstantOutMin=[]  FilterDenConstantOutMax=[]  PCopyOutDataTypeStr=Inherit: Inherit via back propagation  PCopyOutMin=[]  PCopyOutMax=[]  NCopyOutDataTypeStr=Inherit: Inherit via back propagation  NCopyOutMin=[]  NCopyOutMax=[]  IntegratorContinuousStateAttributes=''  IntegratorStateMustResolveToSignalObject=off  IntegratorRTWStateStorageClass=Auto  FilterContinuousStateAttributes=''  FilterStateMustResolveToSignalObject=off  FilterRTWStateStorageClass=Auto  ParallelPVariant=InternalParameters  IdealPVariant=Disabled  IVariant=InternalParameters  DVariant=InternalParameters  IntegratorVariant=Continuous  SatVariant=Disabled  AWVariant=Passthrough  PCopyVariant=Disabled  TRVariant=Disabled  FdbkBlocksVariant=Forward  IdealPFdbkVariant=Disabled  SatFdbkVariant=Disabled  DerivativeFilterVariant=ContFilter  NVariant=InternalParameters  NCopyVariant=Disabled  FilterICVariant=InternalICsFilter  IntegratorICVariant=InternalICs  ExternalResetVariant=Disabled  TRSumVariant=Passthrough  SumFdbkVariant=Disabled  SumVariant=Sum_PID  TsampFilterVariant=InternalTs  TsampNgainVariant=Passthrough  TsampIntegralVariant=Disabled_SignalSpec  ExternalSaturationOutDataTypeStr=Inherit: Same as second input  DerivativeSourceVariant=ErrorSignal  PreIntVariant=InternalPreInt
  PID Controller4 : slpidlib/PID Controller  Commented=on  Controller=PID  Form=Parallel  TimeDomain=Continuous-time  UseExternalTs=off  SampleTime=ControlSampleTime  IntegratorMethod=Forward Euler  FilterMethod=Forward Euler  ControllerParametersSource=internal  P=control.MR.pitchRate_P  I=control.MR.pitchRate_I  UseKiTs=off  D=control.MR.pitchRate_D  UseExternalDerivativeSource=off  N=100  UseFilter=on  TunerSelectOption=Transfer Function Based (PID Tuner App)  InitialConditionSource=internal  InitialConditionForIntegrator=0  InitialConditionForFilter=0  DifferentiatorICPrevScaledInput=0  ExternalReset=none  TrackingMode=off  Kt=1  LimitOutput=on  SatLimitsSource=internal  UpperSaturationLimit=2  LowerSaturationLimit=-2  LinearizeAsGain=on  AntiWindupMode=clamping  Kb=1  LimitIntegrator=off  UpperIntegratorSaturationLimit=inf  LowerIntegratorSaturationLimit=-inf  POutMin=[]  POutMax=[]  IOutMin=[]  IOutMax=[]  DOutMin=[]  DOutMax=[]  NOutMin=[]  NOutMax=[]  SumOutMin=[]  SumOutMax=[]  SaturationOutMin=[]  SaturationOutMax=[]  PParamMin=[]  PParamMax=[]  IParamMin=[]  IParamMax=[]  DParamMin=[]  DParamMax=[]  NParamMin=[]  NParamMax=[]  KbParamMin=[]  KbParamMax=[]  KtParamMin=[]  KtParamMax=[]  KbOutMin=[]  KbOutMax=[]  KtOutMin=[]  KtOutMax=[]  IntegratorOutMin=[]  IntegratorOutMax=[]  FilterOutMin=[]  FilterOutMax=[]  SumI1OutMin=[]  SumI1OutMax=[]  SumI2OutMin=[]  SumI2OutMax=[]  SumI3OutMin=[]  SumI3OutMax=[]  SumI4OutMin=[]  SumI4OutMax=[]  SumDOutMin=[]  SumDOutMax=[]  DifferentiatorOutMin=[]  DifferentiatorOutMax=[]  FilterDiffOutCoefMin=[]  FilterDiffOutCoefMax=[]  ReciprocalOutMin=[]  ReciprocalOutMax=[]  SumDenOutMin=[]  SumDenOutMax=[]  SumNumOutMin=[]  SumNumOutMax=[]  DivideOutMin=[]  DivideOutMax=[]  UdiffTsProdOutMin=[]  UdiffTsProdOutMax=[]  NTsProdOutMin=[]  NTsProdOutMax=[]  UintegralTsProdOutMin=[]  UintegralTsProdOutMax=[]  UngainTsProdOutMin=[]  UngainTsProdOutMax=[]  ClampingZeroOutDataTypeStr=Inherit: Inherit via back propagation  ClampingZeroOutMin=[]  ClampingZeroOutMax=[]  FilterDenConstantOutDataTypeStr=Inherit: Inherit via back propagation  FilterDenConstantOutMin=[]  FilterDenConstantOutMax=[]  PCopyOutDataTypeStr=Inherit: Inherit via back propagation  PCopyOutMin=[]  PCopyOutMax=[]  NCopyOutDataTypeStr=Inherit: Inherit via back propagation  NCopyOutMin=[]  NCopyOutMax=[]  IntegratorContinuousStateAttributes=''  IntegratorStateMustResolveToSignalObject=off  IntegratorRTWStateStorageClass=Auto  FilterContinuousStateAttributes=''  FilterStateMustResolveToSignalObject=off  FilterRTWStateStorageClass=Auto  ParallelPVariant=InternalParameters  IdealPVariant=Disabled  IVariant=InternalParameters  DVariant=InternalParameters  IntegratorVariant=Continuous  SatVariant=Enabled  AWVariant=ContClampingParallel  PCopyVariant=Disabled  TRVariant=Disabled  FdbkBlocksVariant=Forward  IdealPFdbkVariant=Disabled  SatFdbkVariant=Disabled  DerivativeFilterVariant=ContFilter  NVariant=InternalParameters  NCopyVariant=Disabled  FilterICVariant=InternalICsFilter  IntegratorICVariant=InternalICs  ExternalResetVariant=Disabled  TRSumVariant=Passthrough  SumFdbkVariant=Disabled  SumVariant=Sum_PID  TsampFilterVariant=InternalTs  TsampNgainVariant=Passthrough  TsampIntegralVariant=Disabled_SignalSpec  ExternalSaturationOutDataTypeStr=Inherit: Same as second input  DerivativeSourceVariant=ErrorSignal  PreIntVariant=InternalPreInt
  PID Controller6 : slpidlib/PID Controller  Commented=on  Controller=PID  Form=Parallel  TimeDomain=Continuous-time  UseExternalTs=off  SampleTime=ControlSampleTime  IntegratorMethod=Forward Euler  FilterMethod=Forward Euler  ControllerParametersSource=internal  P=control.MR.rollRate_P  I=control.MR.rollRate_I  UseKiTs=off  D=control.MR.rollRate_D  UseExternalDerivativeSource=off  N=100  UseFilter=on  TunerSelectOption=Transfer Function Based (PID Tuner App)  InitialConditionSource=internal  InitialConditionForIntegrator=0  InitialConditionForFilter=0  DifferentiatorICPrevScaledInput=0  ExternalReset=none  TrackingMode=off  Kt=1  LimitOutput=on  SatLimitsSource=internal  UpperSaturationLimit=2  LowerSaturationLimit=-2  LinearizeAsGain=on  AntiWindupMode=clamping  Kb=1  LimitIntegrator=off  UpperIntegratorSaturationLimit=inf  LowerIntegratorSaturationLimit=-inf  POutMin=[]  POutMax=[]  IOutMin=[]  IOutMax=[]  DOutMin=[]  DOutMax=[]  NOutMin=[]  NOutMax=[]  SumOutMin=[]  SumOutMax=[]  SaturationOutMin=[]  SaturationOutMax=[]  PParamMin=[]  PParamMax=[]  IParamMin=[]  IParamMax=[]  DParamMin=[]  DParamMax=[]  NParamMin=[]  NParamMax=[]  KbParamMin=[]  KbParamMax=[]  KtParamMin=[]  KtParamMax=[]  KbOutMin=[]  KbOutMax=[]  KtOutMin=[]  KtOutMax=[]  IntegratorOutMin=[]  IntegratorOutMax=[]  FilterOutMin=[]  FilterOutMax=[]  SumI1OutMin=[]  SumI1OutMax=[]  SumI2OutMin=[]  SumI2OutMax=[]  SumI3OutMin=[]  SumI3OutMax=[]  SumI4OutMin=[]  SumI4OutMax=[]  SumDOutMin=[]  SumDOutMax=[]  DifferentiatorOutMin=[]  DifferentiatorOutMax=[]  FilterDiffOutCoefMin=[]  FilterDiffOutCoefMax=[]  ReciprocalOutMin=[]  ReciprocalOutMax=[]  SumDenOutMin=[]  SumDenOutMax=[]  SumNumOutMin=[]  SumNumOutMax=[]  DivideOutMin=[]  DivideOutMax=[]  UdiffTsProdOutMin=[]  UdiffTsProdOutMax=[]  NTsProdOutMin=[]  NTsProdOutMax=[]  UintegralTsProdOutMin=[]  UintegralTsProdOutMax=[]  UngainTsProdOutMin=[]  UngainTsProdOutMax=[]  ClampingZeroOutDataTypeStr=Inherit: Inherit via back propagation  ClampingZeroOutMin=[]  ClampingZeroOutMax=[]  FilterDenConstantOutDataTypeStr=Inherit: Inherit via back propagation  FilterDenConstantOutMin=[]  FilterDenConstantOutMax=[]  PCopyOutDataTypeStr=Inherit: Inherit via back propagation  PCopyOutMin=[]  PCopyOutMax=[]  NCopyOutDataTypeStr=Inherit: Inherit via back propagation  NCopyOutMin=[]  NCopyOutMax=[]  IntegratorContinuousStateAttributes=''  IntegratorStateMustResolveToSignalObject=off  IntegratorRTWStateStorageClass=Auto  FilterContinuousStateAttributes=''  FilterStateMustResolveToSignalObject=off  FilterRTWStateStorageClass=Auto  ParallelPVariant=InternalParameters  IdealPVariant=Disabled  IVariant=InternalParameters  DVariant=InternalParameters  IntegratorVariant=Continuous  SatVariant=Enabled  AWVariant=ContClampingParallel  PCopyVariant=Disabled  TRVariant=Disabled  FdbkBlocksVariant=Forward  IdealPFdbkVariant=Disabled  SatFdbkVariant=Disabled  DerivativeFilterVariant=ContFilter  NVariant=InternalParameters  NCopyVariant=Disabled  FilterICVariant=InternalICsFilter  IntegratorICVariant=InternalICs  ExternalResetVariant=Disabled  TRSumVariant=Passthrough  SumFdbkVariant=Disabled  SumVariant=Sum_PID  TsampFilterVariant=InternalTs  TsampNgainVariant=Passthrough  TsampIntegralVariant=Disabled_SignalSpec  ExternalSaturationOutDataTypeStr=Inherit: Same as second input  DerivativeSourceVariant=ErrorSignal  PreIntVariant=InternalPreInt
  PID Controller7 : slpidlib/PID Controller  Commented=on  Controller=PID  Form=Parallel  TimeDomain=Continuous-time  UseExternalTs=off  SampleTime=ControlSampleTime  IntegratorMethod=Forward Euler  FilterMethod=Forward Euler  ControllerParametersSource=internal  P=control.MR.yawRate_P  I=control.MR.yawRate_I  UseKiTs=off  D=control.MR.yawRate_D  UseExternalDerivativeSource=off  N=100  UseFilter=on  TunerSelectOption=Transfer Function Based (PID Tuner App)  InitialConditionSource=internal  InitialConditionForIntegrator=0  InitialConditionForFilter=0  DifferentiatorICPrevScaledInput=0  ExternalReset=none  TrackingMode=off  Kt=1  LimitOutput=on  SatLimitsSource=internal  UpperSaturationLimit=2  LowerSaturationLimit=-2  LinearizeAsGain=on  AntiWindupMode=clamping  Kb=1  LimitIntegrator=off  UpperIntegratorSaturationLimit=inf  LowerIntegratorSaturationLimit=-inf  POutMin=[]  POutMax=[]  IOutMin=[]  IOutMax=[]  DOutMin=[]  DOutMax=[]  NOutMin=[]  NOutMax=[]  SumOutMin=[]  SumOutMax=[]  SaturationOutMin=[]  SaturationOutMax=[]  PParamMin=[]  PParamMax=[]  IParamMin=[]  IParamMax=[]  DParamMin=[]  DParamMax=[]  NParamMin=[]  NParamMax=[]  KbParamMin=[]  KbParamMax=[]  KtParamMin=[]  KtParamMax=[]  KbOutMin=[]  KbOutMax=[]  KtOutMin=[]  KtOutMax=[]  IntegratorOutMin=[]  IntegratorOutMax=[]  FilterOutMin=[]  FilterOutMax=[]  SumI1OutMin=[]  SumI1OutMax=[]  SumI2OutMin=[]  SumI2OutMax=[]  SumI3OutMin=[]  SumI3OutMax=[]  SumI4OutMin=[]  SumI4OutMax=[]  SumDOutMin=[]  SumDOutMax=[]  DifferentiatorOutMin=[]  DifferentiatorOutMax=[]  FilterDiffOutCoefMin=[]  FilterDiffOutCoefMax=[]  ReciprocalOutMin=[]  ReciprocalOutMax=[]  SumDenOutMin=[]  SumDenOutMax=[]  SumNumOutMin=[]  SumNumOutMax=[]  DivideOutMin=[]  DivideOutMax=[]  UdiffTsProdOutMin=[]  UdiffTsProdOutMax=[]  NTsProdOutMin=[]  NTsProdOutMax=[]  UintegralTsProdOutMin=[]  UintegralTsProdOutMax=[]  UngainTsProdOutMin=[]  UngainTsProdOutMax=[]  ClampingZeroOutDataTypeStr=Inherit: Inherit via back propagation  ClampingZeroOutMin=[]  ClampingZeroOutMax=[]  FilterDenConstantOutDataTypeStr=Inherit: Inherit via back propagation  FilterDenConstantOutMin=[]  FilterDenConstantOutMax=[]  PCopyOutDataTypeStr=Inherit: Inherit via back propagation  PCopyOutMin=[]  PCopyOutMax=[]  NCopyOutDataTypeStr=Inherit: Inherit via back propagation  NCopyOutMin=[]  NCopyOutMax=[]  IntegratorContinuousStateAttributes=''  IntegratorStateMustResolveToSignalObject=off  IntegratorRTWStateStorageClass=Auto  FilterContinuousStateAttributes=''  FilterStateMustResolveToSignalObject=off  FilterRTWStateStorageClass=Auto  ParallelPVariant=InternalParameters  IdealPVariant=Disabled  IVariant=InternalParameters  DVariant=InternalParameters  IntegratorVariant=Continuous  SatVariant=Enabled  AWVariant=ContClampingParallel  PCopyVariant=Disabled  TRVariant=Disabled  FdbkBlocksVariant=Forward  IdealPFdbkVariant=Disabled  SatFdbkVariant=Disabled  DerivativeFilterVariant=ContFilter  NVariant=InternalParameters  NCopyVariant=Disabled  FilterICVariant=InternalICsFilter  IntegratorICVariant=InternalICs  ExternalResetVariant=Disabled  TRSumVariant=Passthrough  SumFdbkVariant=Disabled  SumVariant=Sum_PID  TsampFilterVariant=InternalTs  TsampNgainVariant=Passthrough  TsampIntegralVariant=Disabled_SignalSpec  ExternalSaturationOutDataTypeStr=Inherit: Same as second input  DerivativeSourceVariant=ErrorSignal  PreIntVariant=InternalPreInt
  Selector1 : Selector  InputPortWidth=3  IndexOptions=Index vector (dialog)  Indices=1  OutputSizes=1
  Selector10 : Selector  Commented=on  InputPortWidth=3  IndexOptions=Index vector (dialog)  Indices=3  OutputSizes=1
  Selector11 : Selector  Commented=on  InputPortWidth=3  IndexOptions=Index vector (dialog)  Indices=1  OutputSizes=1
  Selector12 : Selector  Commented=on  InputPortWidth=3  IndexOptions=Index vector (dialog)  Indices=3  OutputSizes=1
  Selector13 : Selector  Commented=on  InputPortWidth=3  IndexOptions=Index vector (dialog)  Indices=2  OutputSizes=1
  Selector14 : Selector  Commented=on  InputPortWidth=3  IndexOptions=Index vector (dialog)  Indices=2  OutputSizes=1
  Selector15 : Selector  Commented=on  InputPortWidth=3  IndexOptions=Index vector (dialog)  Indices=1  OutputSizes=1
  Selector16 : Selector  Commented=on  InputPortWidth=3  IndexOptions=Index vector (dialog)  Indices=3  OutputSizes=1
  Selector17 : Selector  InputPortWidth=3  IndexOptions=Index vector (dialog)  Indices=3  OutputSizes=1
  Selector2 : Selector  InputPortWidth=3  IndexOptions=Index vector (dialog)  Indices=2  OutputSizes=1
  Selector3 : Selector  InputPortWidth=3  IndexOptions=Index vector (dialog)  Indices=2  OutputSizes=1
  Selector4 : Selector  Commented=on  InputPortWidth=3  IndexOptions=Index vector (dialog)  Indices=2  OutputSizes=1
  Selector5 : Selector  InputPortWidth=3  IndexOptions=Index vector (dialog)  Indices=1  OutputSizes=1
  Selector6 : Selector  InputPortWidth=3  IndexOptions=Index vector (dialog)  Indices=1  OutputSizes=1
  Selector8 : Selector  Commented=on  InputPortWidth=3  IndexOptions=Index vector (dialog)  Indices=1  OutputSizes=1
  Selector9 : Selector  InputPortWidth=3  IndexOptions=Index vector (dialog)  Indices=2  OutputSizes=1
  Subsystem : Subsystem
  Sum : Sum  Inputs=|+-
  Sum2 : Sum  Inputs=|+-
  Sum4 : Sum  Inputs=++|
  Sum6 : Sum  Commented=on  Inputs=|+-
  Sum7 : Sum  Commented=on  Inputs=|+-
  Sum8 : Sum  Commented=on  Inputs=|+-
  To Workspace : ToWorkspace  VariableName=pitch_d  SampleTime=-1
      settings: Save2DSignal=2-D array (concatenate along first dimension)
  To Workspace1 : ToWorkspace  VariableName=pitch  SampleTime=-1
      settings: Save2DSignal=2-D array (concatenate along first dimension)
  Transfer Fcn1 : TransferFcn  Numerator=[5]  Denominator=[1 5]
  Transfer Fcn3 : TransferFcn  Numerator=[5]  Denominator=[1 5]
  u_phi : Outport
  u_theta : Outport  Port=2
  u_psi : Outport  Port=3
  wires:
  Selector2/1 -> [pitch], Sum/2
  Sum/1 -> PID Controller/1  "e_pitch_IINDI"
  Selector9/1 -> Transfer Fcn3/1
  Euler/1 -> [Euler]
  pqr/1 -> [pqr]
  [Euler] -> Selector2/1
  [Euler] -> Selector5/1
  Selector5/1 -> Sum2/2
  Sum2/1 -> PID Controller2/1  "e_roll_IINDI"
  [pqr] -> Subsystem/5(YawRate)
  Euler_d/1 -> [Euler_d]
  [Euler_d] -> Selector1/1
  [Euler_d] -> Selector9/1
  Transfer Fcn3/1 -> [pitch_d], Derivative1/1, Sum/1  "MR_Pitch_d"
  [Euler_d] -> Subsystem/2(Euler_d)
  [Euler] -> Subsystem/3(Euler)
  YawRate_d/1 -> Subsystem/4(YawRate_d)
  Manual/1 -> Subsystem/1(Manual)
  dw/dt/1 -> [dw_dt]
  Selector8/1 -> INDI_p/2(p)
  From11/1 -> Selector8/1
  From9/1 -> Selector4/1
  Selector4/1 -> INDI_q/2(q)
  Selector10/1 -> INDI_r/2(r)
  From13/1 -> Selector10/1
  From14/1 -> INDI in vector form/2(pqr)
  INDI in vector form/1(u_pqr) -> Demux/1
  Demux/2 -> ?
  Demux/1 -> ?
  Demux/3 -> ?
  Mux/1 -> INDI in vector form/1(pqr_d)
  From15/1 -> Selector12/1
  Selector14/1 -> Improved INDI_q/2(q)
  From18/1 -> Selector14/1
  Selector11/1 -> Improved INDI_p/2(p)
  From16/1 -> Selector11/1
  Selector12/1 -> Improved INDI_r/2(r)
  Mux1/1 -> Improved INDI in vector form/1(pqr_d)
  From17/1 -> Improved INDI in vector form/2(pqr)
  Improved INDI in vector form/1(u_pqr) -> Demux1/1
  Transfer Fcn1/1 -> Sum2/1
  Selector1/1 -> Transfer Fcn1/1  "MR_Roll_d"
  PID Controller/1 -> Sum4/2
  [pitch_d] -> Gain/1
  Gain/1 -> To Workspace/1
  [pitch] -> Gain1/1
  Gain1/1 -> To Workspace1/1
  Improved INDI_p1/1(u_phi) -> u_phi/1
  ? -> Sum7/1  "MR_p_d"
  PID Controller4/1 -> ?
  ? -> Sum6/1  "MR_q_d"
  ? -> Sum8/1  "MR_r_d"
  From21/1 -> Selector16/1
  Sum7/1 -> PID Controller6/1
  Selector13/1 -> Sum6/2
  From23/1 -> Selector15/1
  Sum8/1 -> PID Controller7/1
  Selector16/1 -> Sum8/2
  PID Controller6/1 -> ?
  Selector15/1 -> Sum7/2
  PID Controller7/1 -> ?
  Sum6/1 -> PID Controller4/1
  From22/1 -> Selector13/1
  Selector6/1 -> Improved INDI_p1/2(p)
  [pqr] -> Selector6/1
  PID Controller2/1 -> Improved INDI_p1/1(MR_p_d)  "MR_p_d"
  [pqr] -> Selector17/1
  Selector17/1 -> Improved INDI_r1/2(r)
  Selector3/1 -> Improved INDI_q1/2(q)
  [pqr] -> Selector3/1
  Improved INDI_q1/1(u_theta) -> u_theta/1
  Sum4/1 -> Improved INDI_q1/1(MR_q_d)  "MR_q_d"
  Derivative1/1 -> Sum4/1
  Improved INDI_r1/1(u_psi) -> u_psi/1
  Subsystem/1(MR_r_d) -> Improved INDI_r1/1(MR_r_d)  "MR_r_d"

== system Y3Tiltrotor_sim3_IINDI_case2_1/Subsystem/多旋翼模态/Subsystem ==
  DCMbe : Inport
  MR_vx_d : Inport  Port=2
  MR_vy_d : Inport  Port=3
  vz_d : Inport  Port=4
  Demux : Demux  Outputs=3
  Mux : Mux  Inputs=3
  Product : Product  Multiplication=Matrix(*)
  Reshape : Reshape  OutputDimensionality=Column vector (2-D)
  Reshape1 : Reshape
  MR_vfor_d : Outport
  MR_vlat_d : Outport  Port=2
  MR_w_d : Outport  Port=3
  wires:
  Product/1 -> Reshape1/1
  Reshape/1 -> Product/2
  Mux/1 -> Reshape/1
  DCMbe/1 -> Product/1
  MR_vx_d/1 -> Mux/1
  MR_vy_d/1 -> Mux/2
  vz_d/1 -> Mux/3
  Reshape1/1 -> Demux/1
  Demux/1 -> MR_vfor_d/1
  Demux/2 -> MR_vlat_d/1
  Demux/3 -> MR_w_d/1
